simulink model "Top_Level_Controller"  (R2026b)
settings: Solver=VariableStepAuto
undefined symbols (not defined in the file): t_s
libraries: simulink x4, Coding_Libraries x3, mspfiltlib x1, aerolibutil x1, robotmaniplib x1
settings Model: Creator=Janelyn Anderson  LastModifiedBy=Janelyn Anderson

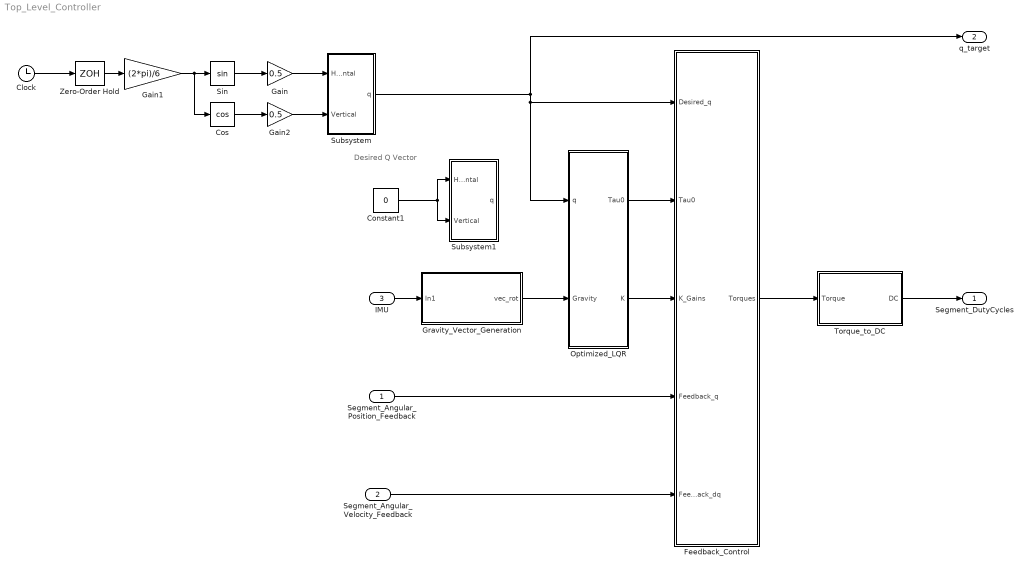
== system Top_Level_Controller ==
  note: Desired Q Vector
  Segment_Angular_Position_Feedback : Inport
  Segment_Angular_Velocity_Feedback : Inport  Port=2
  IMU : Inport  Port=3
  Clock : Clock
  "Constant1 " : Constant  Value=0
  Cos : Trigonometry  Operator=cos
  Feedback_Control : Subsystem
  Gain : Gain  Gain=0.5
  Gain1 : Gain  Gain=(2*pi)/6
  Gain2 : Gain  Gain=0.5
  Gravity_Vector_Generation : Subsystem
  Optimized_LQR : Subsystem
  Sin : Trigonometry
  Subsystem : Subsystem
  Subsystem1 : Subsystem
  Torque_to_DC : Subsystem
  Zero-Order Hold : ZeroOrderHold  SampleTime=t_s
  Segment_DutyCycles : Outport
  q_target : Outport  Port=2
  wires:
  Torque_to_DC/1(DC) -> Segment_DutyCycles/1
  Subsystem/1(q) -> Feedback_Control/1(Desired_q), Optimized_LQR/1(q), q_target/1
  "Constant1 "/1 -> Subsystem1/2(Vertical), Subsystem1/1(Horizontal)
  Gravity_Vector_Generation/1(vec_rot) -> Optimized_LQR/2(Gravity)
  IMU/1 -> Gravity_Vector_Generation/1(In1)
  Optimized_LQR/1(Tau0) -> Feedback_Control/2(Tau0)
  Optimized_LQR/2(K) -> Feedback_Control/3(K_Gains)
  Segment_Angular_Position_Feedback/1 -> Feedback_Control/4(Feedback_q)
  Segment_Angular_Velocity_Feedback/1 -> Feedback_Control/5(Feedback_dq)
  Feedback_Control/1(Torques) -> Torque_to_DC/1(Torque)
  Gain/1 -> Subsystem/1(Horizontal)
  Gain2/1 -> Subsystem/2(Vertical)
  Cos/1 -> Gain2/1
  Zero-Order Hold/1 -> Gain1/1
  Gain1/1 -> Sin/1, Cos/1
  Clock/1 -> Zero-Order Hold/1
  Sin/1 -> Gain/1

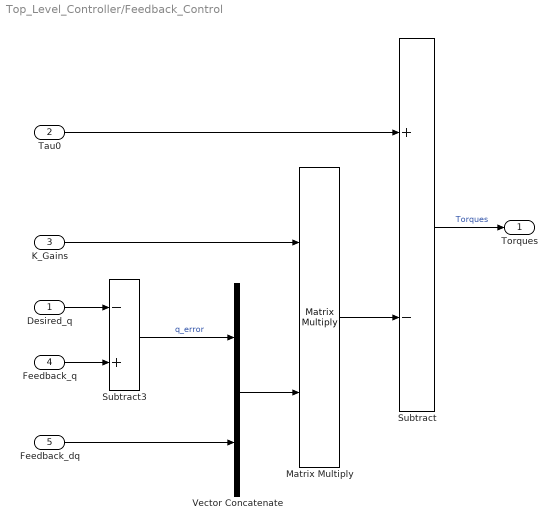
== system Top_Level_Controller/Feedback_Control ==
  Desired_q : Inport
  Tau0 : Inport  Port=2
  K_Gains : Inport  Port=3
  Feedback_q : Inport  Port=4
  Feedback_dq : Inport  Port=5
  Matrix Multiply : Product  Multiplication=Matrix(*)
  Subtract : Sum  Inputs=+-
  Subtract3 : Sum  Inputs=-+
  Vector Concatenate : Concatenate  Mode=Multidimensional array
  Torques : Outport
  wires:
  Feedback_dq/1 -> Vector Concatenate/2
  Desired_q/1 -> Subtract3/1
  Subtract/1 -> Torques/1  "Torques"
  Feedback_q/1 -> Subtract3/2
  Tau0/1 -> Subtract/1
  K_Gains/1 -> Matrix Multiply/1
  Vector Concatenate/1 -> Matrix Multiply/2
  Matrix Multiply/1 -> Subtract/2
  Subtract3/1 -> Vector Concatenate/1  "q_error"

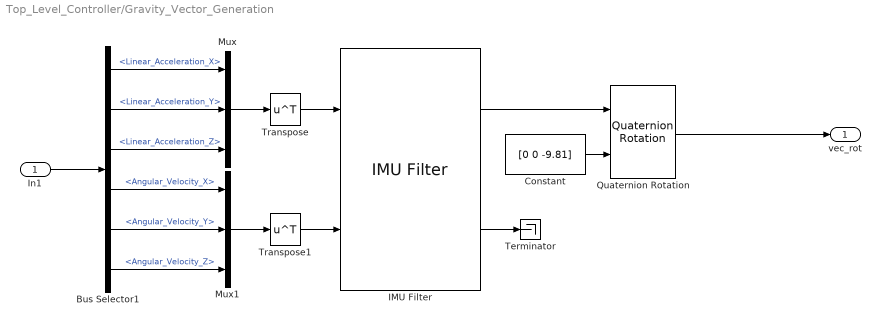
== system Top_Level_Controller/Gravity_Vector_Generation ==
  In1 : Inport
  Bus Selector1 : BusSelector  OutputSignals=Linear_Accleration.Linear_Acceleration_X,Linear_Accleration.Linear_Acceleration_Y,Linear_Accleration.Linear_Acceleration_Z,Angular_Velocity.Angular_Velocity_X,Angular_Velocity.Angular_Velocity_Y,Angular_Velocity.Angular_Velocity_Z
  Constant : Constant  Value=[0 0 -9.81]  VectorParams1D=off
  IMU Filter : mspfiltlib/IMU Filter  DispRefFrame=NED  OrientationFormat=quaternion  DecimationFactor=1  InitialProcessNoise=imufilter.defaultProcessNoise  AccelerometerNoise=0.0001924722*(1/150)  GyroscopeNoise=9.1385e-5*150  GyroscopeDriftNoise=3.0462e-13  LinearAccelerationNoise=0.0096236100000000012  LinearAccelerationDecayFactor=0.01  SimulateUsing=Code generation
  Mux : Mux  Inputs=3
  Mux1 : Mux  Inputs=3
  Quaternion Rotation : aerolibutil/Quaternion Rotation
  Terminator : Terminator
  Transpose : Math  Operator=transpose
  Transpose1 : Math  Operator=transpose
  vec_rot : Outport
  wires:
  In1/1 -> Bus Selector1/1
  Quaternion Rotation/1 -> vec_rot/1
  Bus Selector1/6 -> Mux1/3  "<Angular_Velocity_Z>"
  IMU Filter/2 -> Terminator/1
  Transpose1/1 -> IMU Filter/2
  Mux1/1 -> Transpose1/1
  Bus Selector1/5 -> Mux1/2  "<Angular_Velocity_Y>"
  Bus Selector1/4 -> Mux1/1  "<Angular_Velocity_X>"
  Transpose/1 -> IMU Filter/1
  Bus Selector1/2 -> Mux/2  "<Linear_Acceleration_Y>"
  Bus Selector1/1 -> Mux/1  "<Linear_Acceleration_X>"
  Mux/1 -> Transpose/1
  Bus Selector1/3 -> Mux/3  "<Linear_Acceleration_Z>"
  IMU Filter/1 -> Quaternion Rotation/1
  Constant/1 -> Quaternion Rotation/2

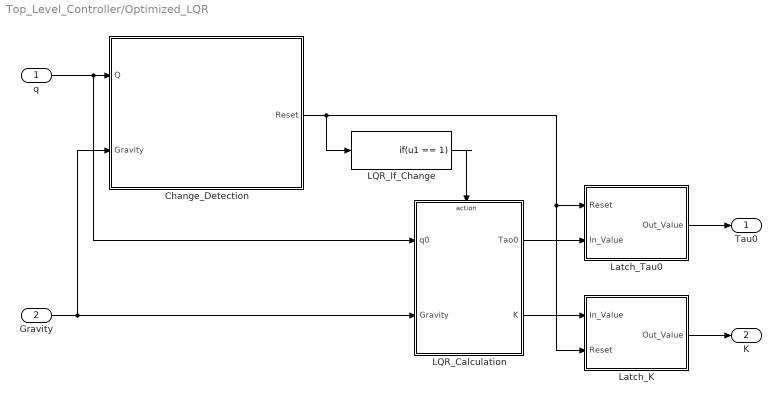
== system Top_Level_Controller/Optimized_LQR ==
  q : Inport
  Gravity : Inport  Port=2
  Change_Detection : Subsystem
  LQR_Calculation : Subsystem  TreatAsAtomicUnit=on
  LQR_If_Change : If  IfExpression=u1 == 1  ShowElse=off
  Latch_K : Subsystem
  Latch_Tau0 : Subsystem
  Tau0 : Outport
  K : Outport  Port=2
  wires:
  Latch_Tau0/1(Out_Value) -> Tau0/1
  Latch_K/1(Out_Value) -> K/1
  LQR_Calculation/1(Tao0) -> Latch_Tau0/2(In_Value)
  Change_Detection/1(Reset) -> Latch_K/2(Reset), Latch_Tau0/1(Reset), LQR_If_Change/1
  q/1 -> LQR_Calculation/1(q0), Change_Detection/1(Q)
  Gravity/1 -> LQR_Calculation/2(Gravity), Change_Detection/2(Gravity)
  LQR_Calculation/2(K) -> Latch_K/1(In_Value)
  LQR_If_Change/1 -> LQR_Calculation/Action

== system Top_Level_Controller/Subsystem ==
  Horizontal : Inport
  Vertical : Inport  Port=2
  Mux1 : Mux  Inputs=6
  Unary Minus : UnaryMinus
  Unary Minus1 : UnaryMinus
  q : Outport
  wires:
  Unary Minus/1 -> Mux1/3
  Mux1/1 -> q/1
  Vertical/1 -> Mux1/6, Unary Minus1/1, Mux1/2
  Horizontal/1 -> Mux1/1, Unary Minus/1, Mux1/5
  Unary Minus1/1 -> Mux1/4

== system Top_Level_Controller/Subsystem1 ==
  Horizontal : Inport
  Vertical : Inport  Port=2
  Mux1 : Mux  Inputs=6
  Unary Minus : UnaryMinus
  Unary Minus1 : UnaryMinus
  q : Outport
  wires:
  Unary Minus/1 -> Mux1/3
  Mux1/1 -> q/1
  Vertical/1 -> Mux1/6, Unary Minus1/1, Mux1/2
  Horizontal/1 -> Mux1/1, Unary Minus/1, Mux1/5
  Unary Minus1/1 -> Mux1/4

== system Top_Level_Controller/Torque_to_DC ==
  Torque : Inport
  Abs1 : Abs  SaturateOnIntegerOverflow=off
  Constant6 : Constant  Value=0
  DC2Torque : Gain  Gain=1.19688
  Gear_Ratio : Gain  Gain=1/10
  Switch4 : Switch  Criteria=u2 > Threshold  Threshold=1e-4  SaturateOnIntegerOverflow=off  InputSameDT=off
  DC : Outport
  wires:
  Torque/1 -> Abs1/1, Switch4/1
  Abs1/1 -> Switch4/2
  DC2Torque/1 -> Gear_Ratio/1
  Constant6/1 -> Switch4/3
  Switch4/1 -> DC2Torque/1
  Gear_Ratio/1 -> DC/1

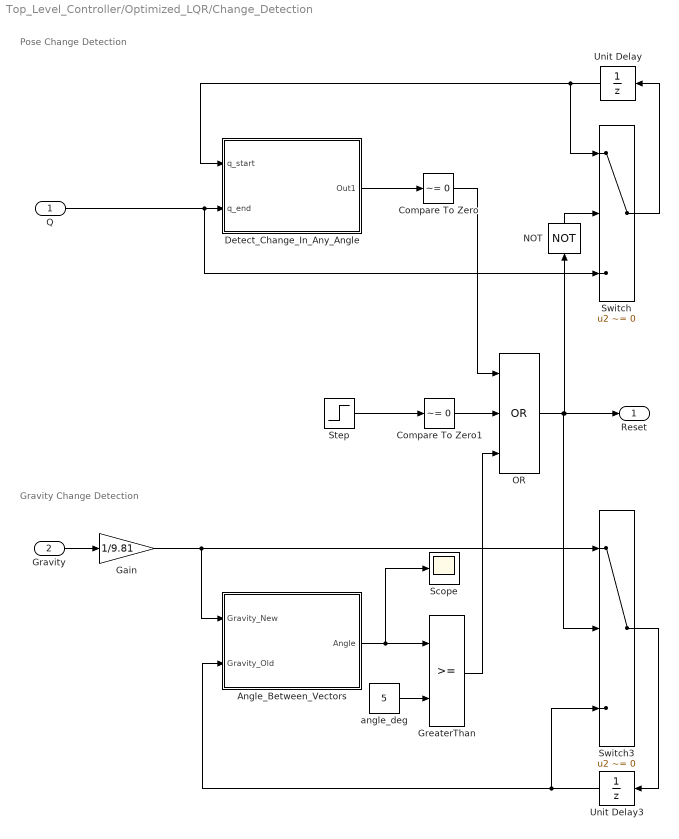
== system Top_Level_Controller/Optimized_LQR/Change_Detection ==
  note: Gravity Change Detection
  note: Pose Change Detection
  Q : Inport
  Gravity : Inport  Port=2
  Angle_Between_Vectors : Subsystem
  Compare To Zero : simulink/Logic and Bit Operations/Compare To Zero  relop=~=  OutDataTypeStr=boolean
  Compare To Zero1 : simulink/Logic and Bit Operations/Compare To Zero  relop=~=  OutDataTypeStr=boolean
  Detect_Change_In_Any_Angle : Subsystem  TreatAsAtomicUnit=on
  Gain : Gain  Gain=1/9.81
  GreaterThan : RelationalOperator  OutDataTypeStr=boolean  RndMeth=Simplest  InputSameDT=off
  NOT : Logic  Operator=NOT  AllPortsSameDT=off  OutDataTypeStr=boolean
  OR : Logic  Operator=OR  Inputs=3  AllPortsSameDT=off  OutDataTypeStr=boolean
  Scope : Scope
      settings: ActiveDisplayYMinimum=-4.4359289646211284  ActiveDisplayYMaximum=8.9205218796962757
  Step : Step  Time=3*t_s  InitialValue=1  FinalValue=0  SampleTime=t_s
  Switch : Switch  Criteria=u2 ~= 0  SaturateOnIntegerOverflow=off  InputSameDT=off
  Switch3 : Switch  Criteria=u2 ~= 0  SaturateOnIntegerOverflow=off  InputSameDT=off
  Unit Delay : UnitDelay  InitialCondition=zeros(1,6)  SampleTime=-1
  Unit Delay3 : UnitDelay  InitialCondition=[0 0 -1]  SampleTime=-1
  angle_deg : Constant  Value=5
  Reset : Outport
  wires:
  Angle_Between_Vectors/1(Angle) -> GreaterThan/1, Scope/1
  Compare To Zero1/1 -> OR/2
  Gravity/1 -> Gain/1
  Unit Delay3/1 -> Angle_Between_Vectors/2(Gravity_Old), Switch3/3
  Switch3/1 -> Unit Delay3/1
  angle_deg/1 -> GreaterThan/2
  Gain/1 -> Switch3/1, Angle_Between_Vectors/1(Gravity_New)
  Step/1 -> Compare To Zero1/1
  GreaterThan/1 -> OR/3
  Compare To Zero/1 -> OR/1
  NOT/1 -> Switch/2
  Unit Delay/1 -> Switch/1, Detect_Change_In_Any_Angle/1(q_start)
  Q/1 -> Detect_Change_In_Any_Angle/2(q_end), Switch/3
  Detect_Change_In_Any_Angle/1(Out1) -> Compare To Zero/1
  Switch/1 -> Unit Delay/1
  OR/1 -> Switch3/2, Reset/1, NOT/1

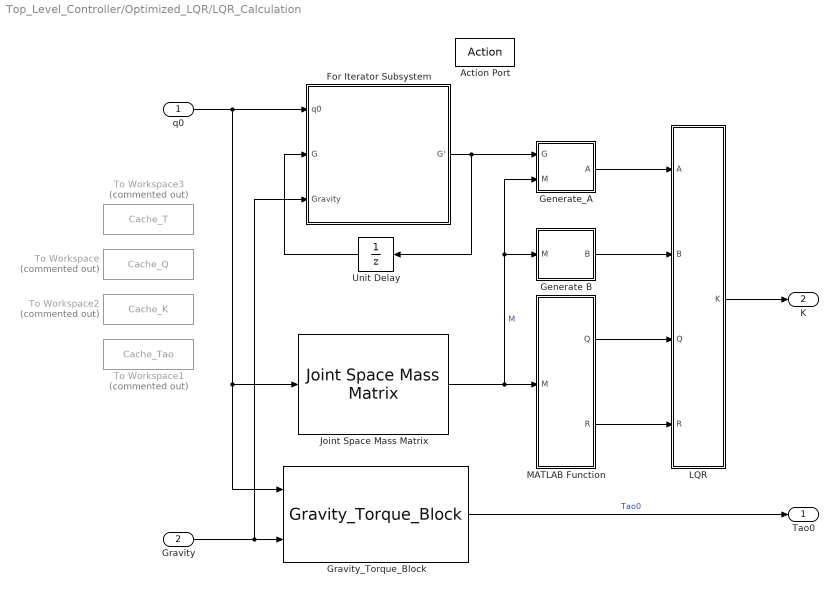
== system Top_Level_Controller/Optimized_LQR/LQR_Calculation ==
  q0 : Inport
  Gravity : Inport  Port=2
  Action Port : ActionPort  PropagateVarSize=During execution
  For Iterator Subsystem : Subsystem  TreatAsAtomicUnit=on
  Generate B : Subsystem
  Generate_A : Subsystem
  Gravity_Torque_Block : Coding_Libraries/Gravity_Torque_Block  RigidBodyTree=Snake_RBT  SimulateUsing=Code generation
  Joint Space Mass Matrix : robotmaniplib/Joint Space Mass Matrix  RigidBodyTree=Snake_RBT  SimulateUsing=Code generation
  LQR : MATLAB Function  TreatAsAtomicUnit=on
  MATLAB Function : MATLAB Function  TreatAsAtomicUnit=on
  To Workspace : ToWorkspace  Commented=on  VariableName=Cache_Q  SaveFormat=Timeseries  SampleTime=1/50
  To Workspace1 : ToWorkspace  Commented=on  VariableName=Cache_Tao  SaveFormat=Timeseries  SampleTime=1/50
  To Workspace2 : ToWorkspace  Commented=on  VariableName=Cache_K  SaveFormat=Timeseries  SampleTime=1/50
  To Workspace3 : ToWorkspace  Commented=on  VariableName=Cache_T  SaveFormat=Timeseries  SampleTime=1/50
  Unit Delay : UnitDelay  InitialCondition=zeros(6)  SampleTime=-1
  Tao0 : Outport
  K : Outport  Port=2
  wires:
  Unit Delay/1 -> For Iterator Subsystem/2(G)
  MATLAB Function/1(Q) -> LQR/3(Q)
  MATLAB Function/2(R) -> LQR/4(R)
  Generate B/1(B) -> LQR/2(B)
  For Iterator Subsystem/1(G') -> Generate_A/1(G), Unit Delay/1
  Generate_A/1(A) -> LQR/1(A)
  Joint Space Mass Matrix/1 -> MATLAB Function/1(M), Generate B/1(M), Generate_A/2(M)  "M"
  LQR/1(K) -> K/1
  Gravity_Torque_Block/1 -> Tao0/1  "Tao0"
  q0/1 -> For Iterator Subsystem/1(q0), Joint Space Mass Matrix/1, Gravity_Torque_Block/1
  Gravity/1 -> Gravity_Torque_Block/2, For Iterator Subsystem/3(Gravity)

== system Top_Level_Controller/Optimized_LQR/Latch_K ==
  In_Value : Inport
  Reset : Inport  Port=2
  Switch1 : Switch  Criteria=u2 ~= 0  SaturateOnIntegerOverflow=off  InputSameDT=off
  Unit Delay1 : UnitDelay  SampleTime=-1
  Out_Value : Outport
  wires:
  In_Value/1 -> Switch1/1
  Unit Delay1/1 -> Switch1/3
  Switch1/1 -> Out_Value/1, Unit Delay1/1  "Tau0"
  Reset/1 -> Switch1/2

== system Top_Level_Controller/Optimized_LQR/Latch_Tau0 ==
  Reset : Inport
  In_Value : Inport  Port=2
  Switch1 : Switch  Criteria=u2 ~= 0  SaturateOnIntegerOverflow=off  InputSameDT=off
  Unit Delay1 : UnitDelay  SampleTime=-1
  Out_Value : Outport
  wires:
  In_Value/1 -> Switch1/1
  Unit Delay1/1 -> Switch1/3
  Switch1/1 -> Out_Value/1, Unit Delay1/1  "Tau0"
  Reset/1 -> Switch1/2

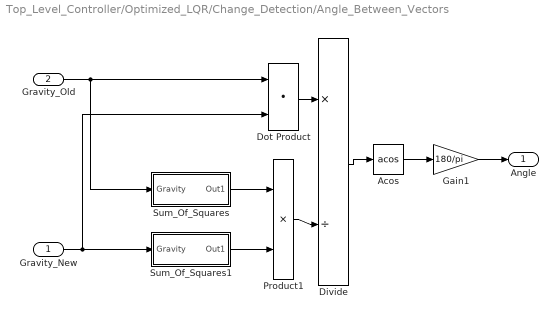
== system Top_Level_Controller/Optimized_LQR/Change_Detection/Angle_Between_Vectors ==
  Gravity_New : Inport
  Gravity_Old : Inport  Port=2
  Acos : Trigonometry  Operator=acos  OutputSignalType=real
  Divide : Product  Inputs=*/
  Dot Product : DotProduct  OutDataTypeStr=Inherit: Inherit via internal rule
  Gain1 : Gain  Gain=180/pi
  Product1 : Product
  Sum_Of_Squares : Subsystem
  Sum_Of_Squares1 : Subsystem
  Angle : Outport
  wires:
  Gain1/1 -> Angle/1
  Sum_Of_Squares1/1(Out1) -> Product1/2
  Gravity_New/1 -> Sum_Of_Squares1/1(Gravity), Dot Product/2
  Gravity_Old/1 -> Sum_Of_Squares/1(Gravity), Dot Product/1
  Sum_Of_Squares/1(Out1) -> Product1/1
  Dot Product/1 -> Divide/1
  Divide/1 -> Acos/1
  Product1/1 -> Divide/2
  Acos/1 -> Gain1/1

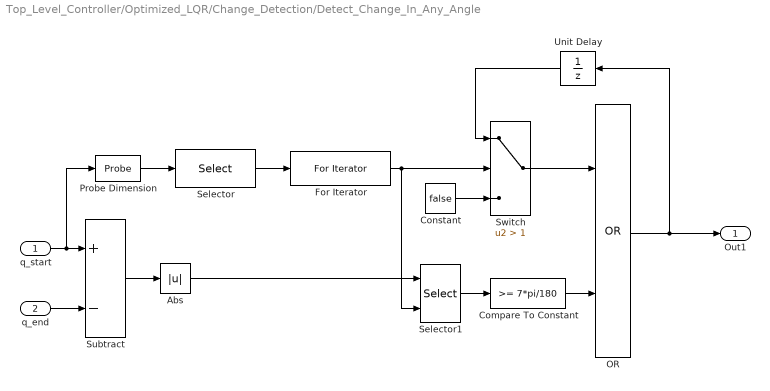
== system Top_Level_Controller/Optimized_LQR/Change_Detection/Detect_Change_In_Any_Angle ==
  q_start : Inport
  q_end : Inport  Port=2
  Abs : Abs  SaturateOnIntegerOverflow=off
  Compare To Constant : simulink/Logic and Bit Operations/Compare To Constant  relop=>=  const=7*pi/180  OutDataTypeStr=boolean
  Constant : Constant  Value=false
  For Iterator : ForIterator  IterationSource=external
  OR : Logic  Operator=OR  AllPortsSameDT=off  OutDataTypeStr=boolean
  Probe Dimension : Probe  ProbeWidth=off  ProbeSampleTime=off  ProbeComplexSignal=off  ProbeSignalDimensions=on
  Selector : Selector  IndexOptions=Index vector (dialog)  Indices=1  OutputSizes=1
  Selector1 : Selector  IndexOptions=Index vector (port)  Indices=[1 3]  OutputSizes=1
  Subtract : Sum  Inputs=+-
  Switch : Switch  Criteria=u2 > Threshold  Threshold=1  SaturateOnIntegerOverflow=off  InputSameDT=off
  Unit Delay : UnitDelay  SampleTime=-1
  Out1 : Outport
  wires:
  Compare To Constant/1 -> OR/2
  Selector1/1 -> Compare To Constant/1
  Abs/1 -> Selector1/1
  Subtract/1 -> Abs/1
  q_end/1 -> Subtract/2
  OR/1 -> Out1/1, Unit Delay/1
  Constant/1 -> Switch/3
  Unit Delay/1 -> Switch/1
  Switch/1 -> OR/1
  For Iterator/1 -> Switch/2, Selector1/2
  Selector/1 -> For Iterator/1
  Probe Dimension/1 -> Selector/1
  q_start/1 -> Probe Dimension/1, Subtract/1

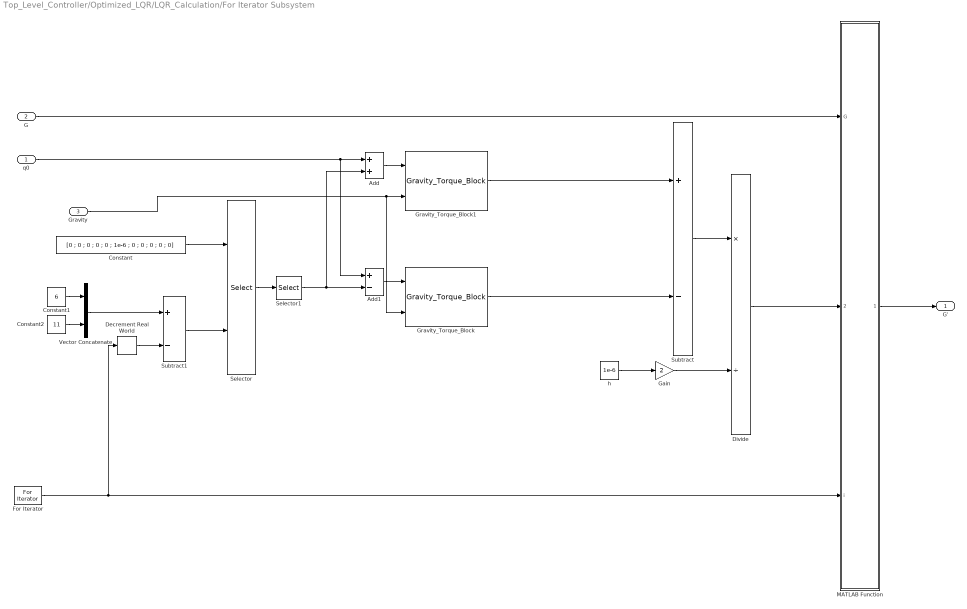
== system Top_Level_Controller/Optimized_LQR/LQR_Calculation/For Iterator Subsystem ==
  q0 : Inport
  G : Inport  Port=2
  Gravity : Inport  Port=3
  Add : Sum
  Add1 : Sum  Inputs=+-
  Constant : Constant  Value=[0 ; 0 ; 0 ; 0 ; 0 ; 1e-6 ; 0 ; 0 ; 0 ; 0 ; 0]  VectorParams1D=off
  Constant1 : Constant  Value=6
  Constant2 : Constant  Value=11
  Decrement Real World : simulink/Additional Math & Discrete/Additional Math: Increment - Decrement/Decrement Real World
  Divide : Product  Inputs=*/
  For Iterator : ForIterator  ResetStates=reset  IterationLimit=6
  Gain : Gain  Gain=2
  Gravity_Torque_Block : Coding_Libraries/Gravity_Torque_Block  RigidBodyTree=Snake_RBT  SimulateUsing=Code generation
  Gravity_Torque_Block1 : Coding_Libraries/Gravity_Torque_Block  RigidBodyTree=Snake_RBT  SimulateUsing=Code generation
  MATLAB Function : MATLAB Function  TreatAsAtomicUnit=on
  Selector : Selector  NumberOfDimensions=2  InputPortWidth=3  IndexOptions=Starting and ending indices (port),Select all  Indices=[1 3],1  OutputSizes=1,1
  Selector1 : Selector  NumberOfDimensions=2  InputPortWidth=3  IndexOptions=Index vector (dialog),Index vector (dialog)  Indices=[1 2 3 4 5 6],1  OutputSizes=1,1
  Subtract : Sum  Inputs=+-
  Subtract1 : Sum  Inputs=+-
  Vector Concatenate : Concatenate
  h : Constant  Value=1e-6
  G' : Outport
  wires:
  Gravity/1 -> Gravity_Torque_Block1/2, Gravity_Torque_Block/2
  G/1 -> MATLAB Function/1(G)
  MATLAB Function/1(G_new) -> G'/1
  For Iterator/1 -> MATLAB Function/3(i), Decrement Real World/1
  Add1/1 -> Gravity_Torque_Block/1
  Add/1 -> Gravity_Torque_Block1/1
  q0/1 -> Add1/1, Add/1
  Gravity_Torque_Block1/1 -> Subtract/1
  Gravity_Torque_Block/1 -> Subtract/2
  Subtract/1 -> Divide/1
  Gain/1 -> Divide/2
  Divide/1 -> MATLAB Function/2(New_Torque)
  h/1 -> Gain/1
  Constant/1 -> Selector/1
  Vector Concatenate/1 -> Subtract1/1
  Constant1/1 -> Vector Concatenate/1
  Constant2/1 -> Vector Concatenate/2
  Subtract1/1 -> Selector/2
  Selector/1 -> Selector1/1
  Selector1/1 -> Add1/2, Add/2
  Decrement Real World/1 -> Subtract1/2

== system Top_Level_Controller/Optimized_LQR/LQR_Calculation/Generate B ==
  M : Inport
  Constant1 : Constant  Value=zeros(6)
  Matrix Divide : Product  Inputs=/  Multiplication=Matrix(*)
  Vector Concatenate2 : Concatenate  Mode=Multidimensional array
  B : Outport
  wires:
  Constant1/1 -> Vector Concatenate2/1
  Vector Concatenate2/1 -> B/1
  M/1 -> Matrix Divide/1
  Matrix Divide/1 -> Vector Concatenate2/2

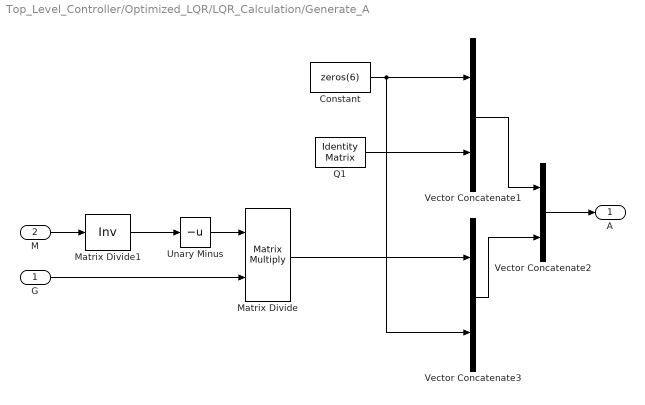
== system Top_Level_Controller/Optimized_LQR/LQR_Calculation/Generate_A ==
  G : Inport
  M : Inport  Port=2
  Constant : Constant  Value=zeros(6)
  Matrix Divide : Product  Inputs=**  Multiplication=Matrix(*)
  Matrix Divide1 : Product  Inputs=/  Multiplication=Matrix(*)
  Q1 : IdentityMatrix  OutputDimensions=6  SampleTime=inf
  Unary Minus : UnaryMinus
  Vector Concatenate1 : Concatenate  Mode=Multidimensional array  ConcatenateDimension=2
  Vector Concatenate2 : Concatenate  Mode=Multidimensional array
  Vector Concatenate3 : Concatenate  Mode=Multidimensional array  ConcatenateDimension=2
  A : Outport
  wires:
  Matrix Divide/1 -> Vector Concatenate3/1
  Q1/1 -> Vector Concatenate1/2
  Vector Concatenate1/1 -> Vector Concatenate2/1
  Vector Concatenate3/1 -> Vector Concatenate2/2
  Vector Concatenate2/1 -> A/1
  Constant/1 -> Vector Concatenate3/2, Vector Concatenate1/1
  G/1 -> Matrix Divide/2
  Unary Minus/1 -> Matrix Divide/1
  Matrix Divide1/1 -> Unary Minus/1
  M/1 -> Matrix Divide1/1

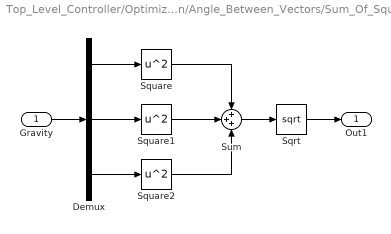
== system Top_Level_Controller/Optimized_LQR/Change_Detection/Angle_Between_Vectors/Sum_Of_Squares ==
  Gravity : Inport
  Demux : Demux  Outputs=3
  Sqrt : Sqrt
  Square : Math  Operator=square
  Square1 : Math  Operator=square
  Square2 : Math  Operator=square
  Sum : Sum  Inputs=+++
  Out1 : Outport
  wires:
  Sqrt/1 -> Out1/1
  Sum/1 -> Sqrt/1
  Square2/1 -> Sum/3
  Square/1 -> Sum/1
  Square1/1 -> Sum/2
  Demux/1 -> Square/1
  Demux/2 -> Square1/1
  Demux/3 -> Square2/1
  Gravity/1 -> Demux/1

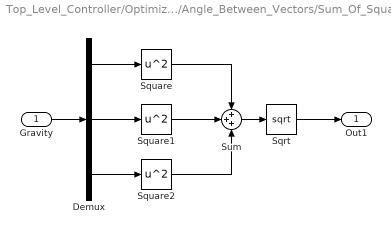
== system Top_Level_Controller/Optimized_LQR/Change_Detection/Angle_Between_Vectors/Sum_Of_Squares1 ==
  Gravity : Inport
  Demux : Demux  Outputs=3
  Sqrt : Sqrt
  Square : Math  Operator=square
  Square1 : Math  Operator=square
  Square2 : Math  Operator=square
  Sum : Sum  Inputs=+++
  Out1 : Outport
  wires:
  Sqrt/1 -> Out1/1
  Sum/1 -> Sqrt/1
  Square2/1 -> Sum/3
  Square/1 -> Sum/1
  Square1/1 -> Sum/2
  Demux/1 -> Square/1
  Demux/2 -> Square1/1
  Demux/3 -> Square2/1
  Gravity/1 -> Demux/1

== matlab function Top_Level_Controller/Optimized_LQR/LQR_Calculation/LQR ==
  data: A input; K output; B input; Q input; R input
function K = fcn(A,B,Q,R)
K = zeros(6, 12);
coder.extrinsic('lqr');
K = lqr(A,B,Q,R);

== matlab function Top_Level_Controller/Optimized_LQR/LQR_Calculation/For Iterator Subsystem/MATLAB Function ==
  data: G input; New_Torque input; G_new output; i input
function G_new = fcn(G, New_Torque, i)

G_new = G;
G_new(:, i) = New_Torque;

== matlab function Top_Level_Controller/Optimized_LQR/LQR_Calculation/MATLAB Function ==
  data: Q output; R output; M input
function [Q,R] = fcn(M)
wn = 20;
Q = blkdiag(wn^4*eye(6), 2*wn^2*eye(6));
R = inv(M)^2;
